simulink model "ascensor_duple_t6"  (R2025b)
settings: Solver=ode23t  StartTime=0.0  StopTime=70  MaxStep=1e-4  RelTol=1e-4
values from neighbouring files (symbols this model uses):
  p = parametros_t6()    [tests.m]
settings Model: Creator=Estudiante USM  LastModifiedBy=Estudiante USM

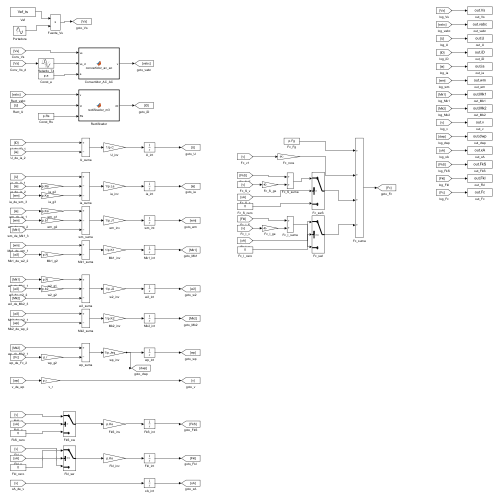
[thumbnail: Simulink's stored preview of the top-level diagram]
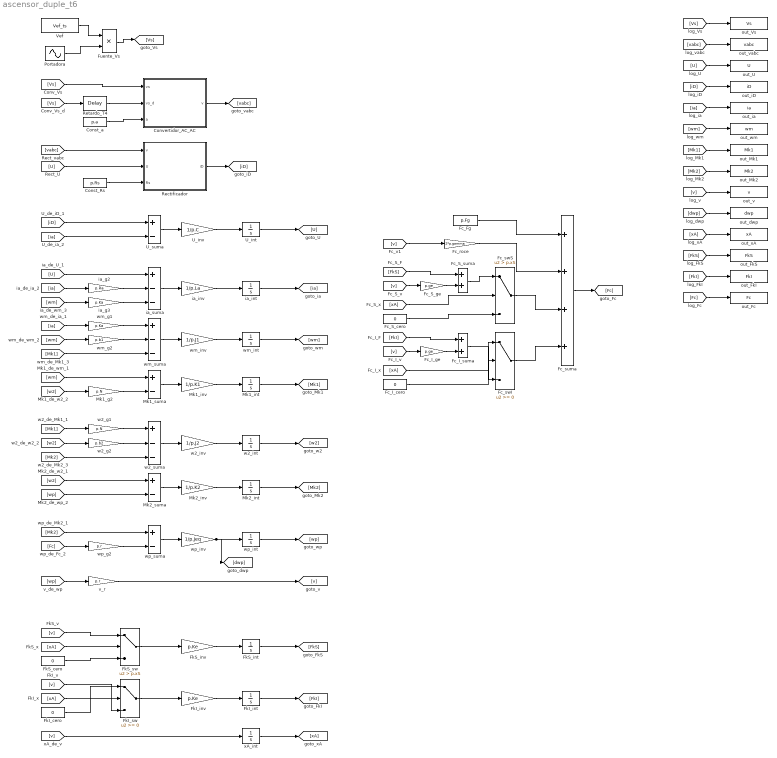
== system ascensor_duple_t6 ==
  Const_Rs : Constant  Value=p.Rs
  Const_a : Constant  Value=p.a
  Convertidor_AC_AC : MATLAB Function  TreatAsAtomicUnit=on
  Fc_Fg : Constant  Value=p.Fg
  Fc_I_cero : Constant  Value=0
  Fc_I_ge : Gain  Gain=p.ge
  Fc_I_suma : Sum
  Fc_S_cero : Constant  Value=0
  Fc_S_ge : Gain  Gain=p.ge
  Fc_S_suma : Sum
  Fc_roce : Gain  Gain=2*p.gamma
  Fc_suma : Sum  Inputs=++++
  Fc_swI : Switch  SaturateOnIntegerOverflow=off  InputSameDT=off
  Fc_swS : Switch  Criteria=u2 > Threshold  Threshold=p.xS  SaturateOnIntegerOverflow=off  InputSameDT=off
  FkI_cero : Constant  Value=0
  FkI_int : Integrator  InitialCondition=p.x0(9)
  FkI_inv : Gain  Gain=p.Ke
  FkI_sw : Switch  SaturateOnIntegerOverflow=off  InputSameDT=off
  FkS_cero : Constant  Value=0
  FkS_int : Integrator  InitialCondition=p.x0(8)
  FkS_inv : Gain  Gain=p.Ke
  FkS_sw : Switch  Criteria=u2 > Threshold  Threshold=p.xS  SaturateOnIntegerOverflow=off  InputSameDT=off
  Fuente_Vs : Product
  Mk1_g2 : Gain  Gain=p.N
  Mk1_int : Integrator  InitialCondition=p.x0(4)
  Mk1_inv : Gain  Gain=1/p.K1
  Mk1_suma : Sum  Inputs=+-
  Mk2_int : Integrator  InitialCondition=p.x0(6)
  Mk2_inv : Gain  Gain=1/p.K2
  Mk2_suma : Sum  Inputs=+-
  Portadora : Sin  Amplitude=sqrt(2)  Frequency=2*pi*p.f  SampleTime=0
  Rectificador : MATLAB Function  TreatAsAtomicUnit=on
  Retardo_T4 : TransportDelay  DelayTime=1/(4*p.f)  BufferSize=4096
  U_int : Integrator  InitialCondition=p.x0(1)
  U_inv : Gain  Gain=1/p.C
  U_suma : Sum  Inputs=+-
  Vef : FromWorkspace  VariableName=Vef_ts  OutputAfterFinalValue=Holding final value
  ia_g2 : Gain  Gain=p.Ra
  ia_g3 : Gain  Gain=p.Ka
  ia_int : Integrator  InitialCondition=p.x0(2)
  ia_inv : Gain  Gain=1/p.La
  ia_suma : Sum  Inputs=+--
  out_Fc : ToWorkspace  VariableName=Fc  SaveFormat=Timeseries  SampleTime=p.Ts_log
  out_FkI : ToWorkspace  VariableName=FkI  SaveFormat=Timeseries  SampleTime=p.Ts_log
  out_FkS : ToWorkspace  VariableName=FkS  SaveFormat=Timeseries  SampleTime=p.Ts_log
  out_Mk1 : ToWorkspace  VariableName=Mk1  SaveFormat=Timeseries  SampleTime=p.Ts_log
  out_Mk2 : ToWorkspace  VariableName=Mk2  SaveFormat=Timeseries  SampleTime=p.Ts_log
  out_U : ToWorkspace  VariableName=U  SaveFormat=Timeseries  SampleTime=p.Ts_log
  out_Vs : ToWorkspace  VariableName=Vs  SaveFormat=Timeseries  SampleTime=p.Ts_log
  out_dwp : ToWorkspace  VariableName=dwp  SaveFormat=Timeseries  SampleTime=p.Ts_log
  out_iD : ToWorkspace  VariableName=iD  SaveFormat=Timeseries  SampleTime=p.Ts_log
  out_ia : ToWorkspace  VariableName=ia  SaveFormat=Timeseries  SampleTime=p.Ts_log
  out_v : ToWorkspace  VariableName=v  SaveFormat=Timeseries  SampleTime=p.Ts_log
  out_vabc : ToWorkspace  VariableName=vabc  SaveFormat=Timeseries  SampleTime=p.Ts_log
  out_wm : ToWorkspace  VariableName=wm  SaveFormat=Timeseries  SampleTime=p.Ts_log
  out_xA : ToWorkspace  VariableName=xA  SaveFormat=Timeseries  SampleTime=p.Ts_log
  v_r : Gain  Gain=p.r
  w2_g1 : Gain  Gain=p.N
  w2_g2 : Gain  Gain=p.b2
  w2_int : Integrator  InitialCondition=p.x0(5)
  w2_inv : Gain  Gain=1/p.J2
  w2_suma : Sum  Inputs=+--
  wm_g1 : Gain  Gain=p.Ka
  wm_g2 : Gain  Gain=p.b1
  wm_int : Integrator  InitialCondition=p.x0(3)
  wm_inv : Gain  Gain=1/p.J1
  wm_suma : Sum  Inputs=+--
  wp_g2 : Gain  Gain=p.r
  wp_int : Integrator  InitialCondition=p.x0(7)
  wp_inv : Gain  Gain=1/p.Jeq
  wp_suma : Sum  Inputs=+-
  xA_int : Integrator  InitialCondition=p.x0(10)
  wires:
  Vef/1 -> Fuente_Vs/1
  Portadora/1 -> Fuente_Vs/2
  Fuente_Vs/1 -> [Vs]
  [Vs] -> Retardo_T4/1
  [Vs] -> Convertidor_AC_AC/1(vs)
  Retardo_T4/1 -> Convertidor_AC_AC/2(vs_d)
  Const_a/1 -> Convertidor_AC_AC/3(a)
  Convertidor_AC_AC/1(v) -> [vabc]
  [vabc] -> Rectificador/1(v)
  [U] -> Rectificador/2(U)
  Const_Rs/1 -> Rectificador/3(Rs)
  Rectificador/1(iD) -> [iD]
  [iD] -> U_suma/1
  [ia] -> U_suma/2
  U_suma/1 -> U_inv/1
  U_inv/1 -> U_int/1
  U_int/1 -> [U]
  [U] -> ia_suma/1
  [ia] -> ia_g2/1
  ia_g2/1 -> ia_suma/2
  [wm] -> ia_g3/1
  ia_g3/1 -> ia_suma/3
  ia_suma/1 -> ia_inv/1
  ia_inv/1 -> ia_int/1
  ia_int/1 -> [ia]
  [ia] -> wm_g1/1
  wm_g1/1 -> wm_suma/1
  [wm] -> wm_g2/1
  wm_g2/1 -> wm_suma/2
  [Mk1] -> wm_suma/3
  wm_suma/1 -> wm_inv/1
  wm_inv/1 -> wm_int/1
  wm_int/1 -> [wm]
  [wm] -> Mk1_suma/1
  [w2] -> Mk1_g2/1
  Mk1_g2/1 -> Mk1_suma/2
  Mk1_suma/1 -> Mk1_inv/1
  Mk1_inv/1 -> Mk1_int/1
  Mk1_int/1 -> [Mk1]
  [Mk1] -> w2_g1/1
  w2_g1/1 -> w2_suma/1
  [w2] -> w2_g2/1
  w2_g2/1 -> w2_suma/2
  [Mk2] -> w2_suma/3
  w2_suma/1 -> w2_inv/1
  w2_inv/1 -> w2_int/1
  w2_int/1 -> [w2]
  [w2] -> Mk2_suma/1
  [wp] -> Mk2_suma/2
  Mk2_suma/1 -> Mk2_inv/1
  Mk2_inv/1 -> Mk2_int/1
  Mk2_int/1 -> [Mk2]
  [Mk2] -> wp_suma/1
  [Fc] -> wp_g2/1
  wp_g2/1 -> wp_suma/2
  wp_suma/1 -> wp_inv/1
  wp_inv/1 -> wp_int/1, [dwp]
  wp_int/1 -> [wp]
  [wp] -> v_r/1
  v_r/1 -> [v]
  [v] -> FkS_sw/1
  FkS_cero/1 -> FkS_sw/3
  [xA] -> FkS_sw/2
  FkS_sw/1 -> FkS_inv/1
  FkS_inv/1 -> FkS_int/1
  FkS_int/1 -> [FkS]
  FkI_cero/1 -> FkI_sw/1
  [v] -> FkI_sw/3
  [xA] -> FkI_sw/2
  FkI_sw/1 -> FkI_inv/1
  FkI_inv/1 -> FkI_int/1
  FkI_int/1 -> [FkI]
  [v] -> xA_int/1
  xA_int/1 -> [xA]
  [v] -> Fc_roce/1
  [FkS] -> Fc_S_suma/1
  [v] -> Fc_S_ge/1
  Fc_S_ge/1 -> Fc_S_suma/2
  Fc_S_suma/1 -> Fc_swS/1
  Fc_S_cero/1 -> Fc_swS/3
  [xA] -> Fc_swS/2
  [FkI] -> Fc_I_suma/1
  [v] -> Fc_I_ge/1
  Fc_I_ge/1 -> Fc_I_suma/2
  Fc_I_cero/1 -> Fc_swI/1
  Fc_I_suma/1 -> Fc_swI/3
  [xA] -> Fc_swI/2
  Fc_Fg/1 -> Fc_suma/1
  Fc_roce/1 -> Fc_suma/2
  Fc_swS/1 -> Fc_suma/3
  Fc_swI/1 -> Fc_suma/4
  Fc_suma/1 -> [Fc]
  [Vs] -> out_Vs/1
  [vabc] -> out_vabc/1
  [U] -> out_U/1
  [iD] -> out_iD/1
  [ia] -> out_ia/1
  [wm] -> out_wm/1
  [Mk1] -> out_Mk1/1
  [Mk2] -> out_Mk2/1
  [v] -> out_v/1
  [dwp] -> out_dwp/1
  [xA] -> out_xA/1
  [FkS] -> out_FkS/1
  [FkI] -> out_FkI/1
  [Fc] -> out_Fc/1

== matlab function ascensor_duple_t6/Convertidor_AC_AC ==
  data: vs input; v output; vs_d input; a input
function v = convertidor_ac_ac(vs, vs_d, a)
% Convertidor ideal 1F -> 3F: vs = alfa, vs_d = Vs(t - T/4) = beta
v = a*[vs; -0.5*vs + (sqrt(3)/2)*vs_d; -0.5*vs - (sqrt(3)/2)*vs_d];
end

== matlab function ascensor_duple_t6/Rectificador ==
  data: v input; iD output; U input; Rs input
function iD = rectificador_m3(v, U, Rs)
% Corriente total de los diodos que conducen hacia el bus de tension U
iD = 0;
for k = 1:3
    if v(k) > U
        iD = iD + (v(k) - U)/Rs;
    end
end
end
